simulink model "exampleResponse"  (R2021b)
settings: Solver=VariableStepAuto  StartTime=0.0  StopTime=10  RelTol=1e-3
libraries: uavalgslib x1
settings Model: Creator=jihoo  LastModifiedBy=jihoo

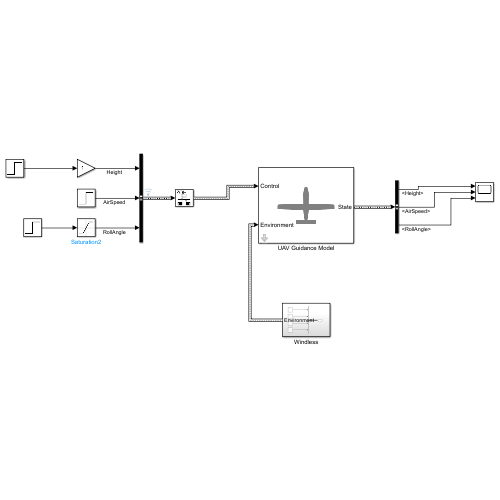
[thumbnail: Simulink's stored preview of the top-level diagram]
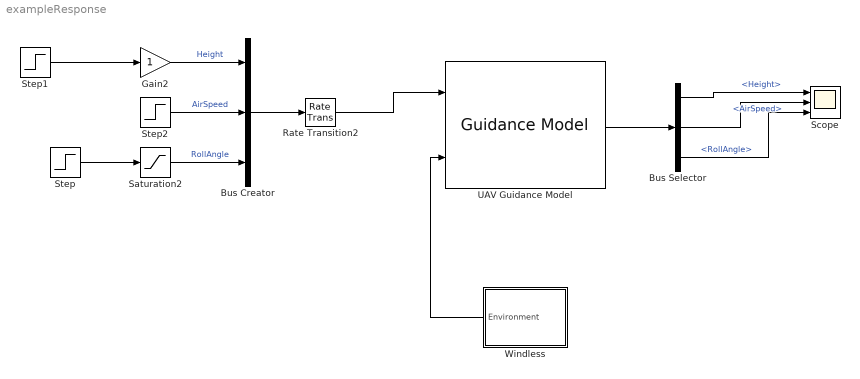
== system exampleResponse ==
  Bus Creator : BusCreator  Inputs=3  OutDataTypeStr=Bus: FixedWingControlBus  NonVirtualBus=on
  Bus Selector : BusSelector  OutputSignals=Height,AirSpeed,RollAngle
  Gain2 : Gain
  Rate Transition2 : RateTransition  OutPortSampleTime=0.1
  Saturation2 : Saturate  UpperLimit=20/180*pi  LowerLimit=-20/180*pi
  Scope : Scope  NumInputPorts=3
  Step : Step  SampleTime=0
  Step1 : Step  SampleTime=0
  Step2 : Step  SampleTime=0
  UAV Guidance Model : uavalgslib/Guidance Model  ModelType=FixedWingGuidance  SpecifiedDataType=double  SimulateUsing=Code generation  InitialWorldPositionMultirotor=[0; 0; 0]  InitialWorldVelocityMultirotor=[0; 0; 0]  InitialEulerZYXMultirotor=[0; 0; 0]  InitialBodyAngularRateRPYMultirotor=[0; 0; 0]  InitialThrustMultirotor=0  InitialNorthFixedWing=0  InitialEastFixedWing=0  InitialHeightFixedWing=0  InitialAirSpeedFixedWing=15  InitialHeadingAngleFixedWing=0  InitialFlightPathAngleFixedWing=0  InitialRollAngleFixedWing=0  InitialRollAngleRateFixedWing=0  PDRollMultirotor=[3402.97,116.67]  PDPitchMultirotor=[3402.97, 116.67]  PYawRateMultirotor=1950  PThrustMultirotor=3900  MassMultirotor=0.1  PHeightFixedWing=3.9  PHeadingAngleFixedWing=3.9  PFlightPathAngleFixedWing=39  PDRollFixedWing=[5.9414, 3.9]  PAirSpeedFixedWing=1  FlightPathAngleLimitsFixedWing=[-pi/6, pi/6]  StateBusName='FixedWingStateBus'  ControlBusName='FixedWingControlBus'  EnvironmentBusName='FixedWingEnvironmentBus'  DataType=double
      settings: SourceProductBaseCode=UV
  Windless : Subsystem  VariantControl=NoWind
  wires:
  Bus Selector/1 -> Scope/1  "<Height>"
  Bus Selector/2 -> Scope/2  "<AirSpeed>"
  Bus Selector/3 -> Scope/3  "<RollAngle>"
  Step2/1 -> Bus Creator/2  "AirSpeed"
  Step/1 -> Saturation2/1
  Gain2/1 -> Bus Creator/1  "Height"
  Saturation2/1 -> Bus Creator/3  "RollAngle"
  Rate Transition2/1 -> UAV Guidance Model/1
  Bus Creator/1 -> Rate Transition2/1
  Step1/1 -> Gain2/1
  UAV Guidance Model/1 -> Bus Selector/1
  Windless/1(Environment) -> UAV Guidance Model/2

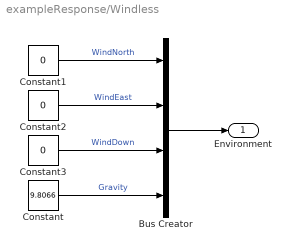
== system exampleResponse/Windless ==
  Bus Creator : BusCreator  Inputs=4  OutDataTypeStr=Bus: FixedWingEnvironmentBus  NonVirtualBus=on
  Constant : Constant  Value=9.8066
  Constant1 : Constant  Value=0
  Constant2 : Constant  Value=0
  Constant3 : Constant  Value=0
  Environment : Outport  VectorParamsAs1DForOutWhenUnconnected=off
  wires:
  Constant/1 -> Bus Creator/4  "Gravity"
  Bus Creator/1 -> Environment/1
  Constant1/1 -> Bus Creator/1  "WindNorth"
  Constant3/1 -> Bus Creator/3  "WindDown"
  Constant2/1 -> Bus Creator/2  "WindEast"
